simulink library "Vehicle_Inputs"  (R2025a)
settings: Solver=VariableStepAuto  StartTime=0.0  StopTime=10.0  RelTol=1e-3
values from neighbouring files (symbols this model uses):
  b = beta    [frameRotationXYextr.m]
libraries: Damper_Control_Axle2 x2, Vehicle_Outputs x2, simulink x2, Spring_Control_Axle2 x1, Damper_Control_Axle3 x1, Spring_Control_Axle3 x1, sim3dlib x1, Tire_Utilities x1
Description:
  | Simscape Vehicle Templates Library
  | 
  | Copyright 2018-2026 The MathWorks, Inc.
settings Model: Creator=smiller  LastModifiedBy=smiller
settings OptimizationCC: ReuseModelBlockBuffer=off
settings ModelReferenceCC: EnableRefExpFcnMdlSchedulingChecks=on
settings RTWCC: GPUComputeCapability=3.5

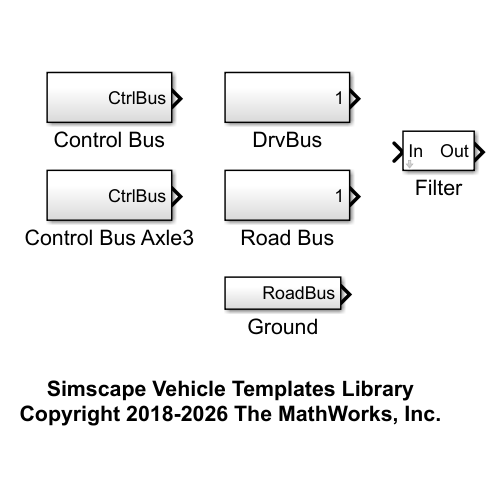
[thumbnail: Simulink's stored preview of the top-level diagram]
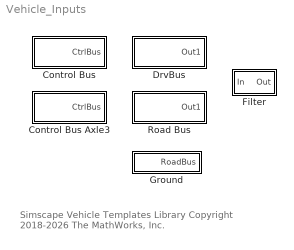
== system Vehicle_Inputs ==
  note: Simscape Vehicle Templates Library
      | Copyright 2018-2026 The MathWorks, Inc.
  Control Bus : Subsystem
  Control Bus Axle3 : Subsystem
  DrvBus : Subsystem
  Filter : Subsystem  mask(First-order lag supporting vector signals){b=b, x_initial=[0 0 0 0]}
      mask prompts: b "Filter time constant"; x_initial "Initial output"
      mask help: Models a lag of the form 1/(b*s+1) where s is the Laplace operator.
  Ground : Subsystem
  Road Bus : Subsystem

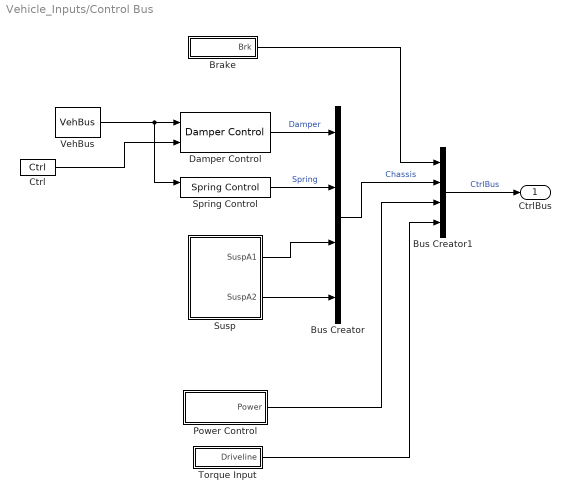
== system Vehicle_Inputs/Control Bus ==
  Brake : Subsystem  mask{brake_on_time=10}
      mask prompts: brake_on_time "Brake On Time (sec)"
      mask TypeOptions brake_on_time: Step/Time
  Bus Creator : BusCreator  Inputs=4
  Bus Creator1 : BusCreator  Inputs=4
  Ctrl : Damper_Control_Axle2/Ctrl  SystemSampleTime=-1  VariantActivationTime=update diagram  EmptyChoice=off  PassThrough=off  PassThroughVariantControl=(default)  EmptyChoiceVariantControl=(default)  AllowFlexibleInterface=on  Latency=0  AutoFrameSizeCalculation=off
  Damper Control : Damper_Control_Axle2/Damper Control  popup_damper_control_A1=Coefficient  popup_damper_control_A2=Coefficient
  Power Control : Subsystem
  Spring Control : Spring_Control_Axle2/Spring Control  VariantControl=Choice  popup_spring_control_A1=None  popup_gas_spring_A1=Stiff  popup_spring_control_A2=None  popup_gas_spring_A2=Stiff
      settings: AttributesFormatString=%<popup_spring_control>
  Susp : Subsystem
  Torque Input : Subsystem  mask{popup_torque_input=Low Torque, Rear}
      mask prompts: popup_torque_input "Maneuver Torque"
      mask init:
      | if (popup_torque_input == 1)
      |     torque_ra = 200*2*2*2;
      |     torque_fa = 0;
      | elseif (popup_torque_input == 2)
      |     torque_ra = 0;
      |     torque_fa = 200*2*2*2;
      | elseif (popup_torque_input == 3)
      |     torque_ra = 200*2;
      |     torque_fa = 0;
      | elseif (popup_torque_input == 4)
      |     torque_ra = 0;
      |     torque_fa = 200*2;
      | elseif (popup_torque_input == 5)
      |     torque_ra = 0;
      |     torque_fa = 0;
      | end
      mask TypeOptions popup_torque_input: Full Torque, Rear | Full Torque, Front | Low Torque, Rear | Low Torque, Front | None
  VehBus : Vehicle_Outputs/VehBus  SystemSampleTime=-1  VariantActivationTime=update diagram  EmptyChoice=off  PassThrough=off  PassThroughVariantControl=(default)  EmptyChoiceVariantControl=(default)  AllowFlexibleInterface=on  Latency=0  AutoFrameSizeCalculation=off
  CtrlBus : Outport  VectorParamsAs1DForOutWhenUnconnected=off
  wires:
  Power Control/1(Power) -> Bus Creator1/3
  Bus Creator/1 -> Bus Creator1/2  "Chassis"
  Torque Input/1(Driveline) -> Bus Creator1/4
  Brake/1(Brk) -> Bus Creator1/1
  Bus Creator1/1 -> CtrlBus/1  "CtrlBus"
  Susp/2(SuspA2) -> Bus Creator/4
  Susp/1(SuspA1) -> Bus Creator/3
  VehBus/1 -> Spring Control/1, Damper Control/1
  Damper Control/1 -> Bus Creator/1  "Damper"
  Spring Control/1 -> Bus Creator/2  "Spring"
  Ctrl/1 -> Damper Control/2

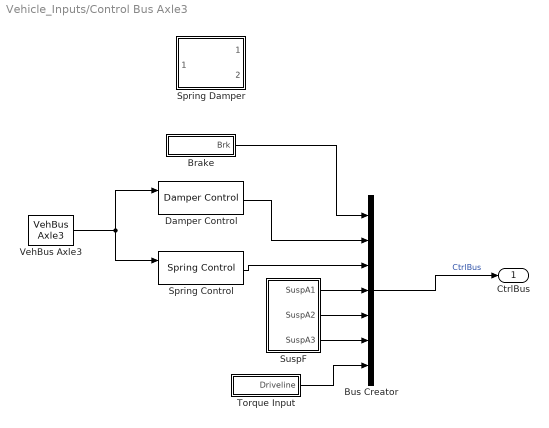
== system Vehicle_Inputs/Control Bus Axle3 ==
  Brake : Subsystem  mask{brake_on_time=10}
      mask prompts: brake_on_time "Brake On Time (sec)"
      mask TypeOptions brake_on_time: Step/Time
  Bus Creator : BusCreator  Inputs=7
  Damper Control : Damper_Control_Axle3/Damper Control  VariantControl=Choice  popup_damper_control_A1=None  popup_damper_control_A2=None  popup_damper_control_A3=None
      settings: AttributesFormatString=%<popup_damper_control>
  Spring Control : Spring_Control_Axle3/Spring Control  VariantControl=Choice  popup_spring_control_A1=None  popup_spring_control_A2=None  popup_spring_control_A3=None
      settings: AttributesFormatString=%<popup_spring_control>
  Spring Damper : Subsystem
  SuspF : Subsystem
  Torque Input : Subsystem  mask{popup_torque_input=Low Torque, Rear}
      mask prompts: popup_torque_input "Maneuver Torque"
      mask init: same as Vehicle_Inputs/Control Bus/Torque Input
      mask TypeOptions popup_torque_input: Full Torque, Rear | Full Torque, Front | Low Torque, Rear | Low Torque, Front | None
  VehBus Axle3 : Vehicle_Outputs/VehBus Axle3  SystemSampleTime=-1  VariantActivationTime=update diagram  EmptyChoice=off  PassThrough=off  PassThroughVariantControl=(default)  EmptyChoiceVariantControl=(default)  AllowFlexibleInterface=on  Latency=0  AutoFrameSizeCalculation=off
  CtrlBus : Outport  VectorParamsAs1DForOutWhenUnconnected=off
  wires:
  SuspF/3(SuspA3) -> Bus Creator/6
  SuspF/1(SuspA1) -> Bus Creator/4
  SuspF/2(SuspA2) -> Bus Creator/5
  Bus Creator/1 -> CtrlBus/1  "CtrlBus"
  Spring Control/1 -> Bus Creator/3
  Damper Control/1 -> Bus Creator/2
  Brake/1(Brk) -> Bus Creator/1
  Torque Input/1(Driveline) -> Bus Creator/7
  VehBus Axle3/1 -> Spring Control/1, Damper Control/1

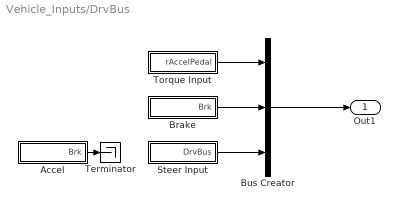
== system Vehicle_Inputs/DrvBus ==
  Accel : Subsystem  mask{brake_on_time=10}
      mask prompts: brake_on_time "Brake On Time (sec)"
      mask TypeOptions brake_on_time: Step/Time
  Brake : Subsystem  mask{brake_on_time=10}
      mask prompts: brake_on_time "Brake On Time (sec)"
      mask TypeOptions brake_on_time: Step/Time
  Bus Creator : BusCreator  Inputs=3
  Steer Input : Subsystem  mask{popup_steer_input=Sequence}
      mask prompts: popup_steer_input "Steer Input"
      mask TypeOptions popup_steer_input: Straight | Step | Sequence | Lane Change
  Terminator : Terminator
  Torque Input : Subsystem  mask{popup_torque_input=Full Torque}
      mask prompts: popup_torque_input "Maneuver Torque"
      mask init:
      | if (popup_torque_input == 1)
      |     rPedalValue = 1;
      | elseif (popup_torque_input == 2)
      |     rPedalValue = 0.25;
      | elseif (popup_torque_input == 3)
      |     rPedalValue = 0;
      | end
      mask TypeOptions popup_torque_input: Full Torque | Low Torque | None
  Out1 : Outport  VectorParamsAs1DForOutWhenUnconnected=off
  wires:
  Accel/1(Brk) -> Terminator/1
  Torque Input/1(rAccelPedal) -> Bus Creator/1
  Brake/1(Brk) -> Bus Creator/2
  Bus Creator/1 -> Out1/1
  Steer Input/1(DrvBus) -> Bus Creator/3

== system Vehicle_Inputs/Filter ==
  In : Inport
  Gain : Gain  Gain=1/b
  Integrator : Integrator  InitialCondition=x_initial*b
  Sum : Sum  Inputs=|+-  InputSameDT=on  SaturateOnIntegerOverflow=on  OutDataTypeStr=Inherit: Same as first input
  Out : Outport  VectorParamsAs1DForOutWhenUnconnected=off
  wires:
  Sum/1 -> Integrator/1
  In/1 -> Sum/1
  Integrator/1 -> Gain/1
  Gain/1 -> Sum/2, Out/1

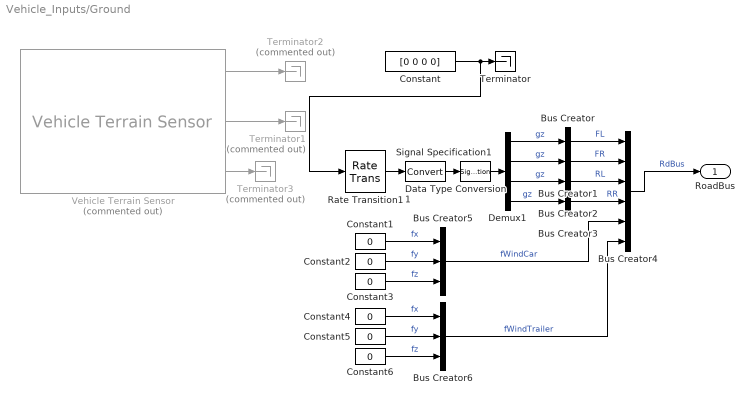
== system Vehicle_Inputs/Ground ==
  Bus Creator{,1..3} (4 alike) : BusCreator  Inputs=1
  Bus Creator4 : BusCreator  Inputs=6
  Bus Creator5 : BusCreator  Inputs=3
  Bus Creator6 : BusCreator  Inputs=3
  Constant : Constant  Value=[0 0 0 0]
  Constant{1..6} (6 alike) : Constant  Value=0
  Data Type Conversion1 : DataTypeConversion  SaturateOnIntegerOverflow=off  RndMeth=Floor
  Demux1 : Demux
  Rate Transition1 : RateTransition
  Signal Specification1 : SignalSpecification  Unit=m
  Terminator : Terminator
  Terminator1 : Terminator  Commented=on
  Terminator2 : Terminator  Commented=on
  Terminator3 : Terminator  Commented=on
  Vehicle Terrain Sensor : sim3dlib/Vehicle Terrain Sensor  Commented=on  ActorTag=SimulinkActor1  VehExtEn=Constant  TireRadiiExt=Constant  VehCntrLngthVal=0  TireRadiiVal=.55  VehRayLngth=5  LfRayLngth=5  RfRayLngth=5  LrRayLngth=5  RrRayLngth=5  VehRayOffset=0  LfRayOffset=0  RfRayOffset=0  LrRayOffset=0  RrRayOffset=0  VehEn=on  LfEn=on  RfEn=on  LrEn=on  RrEn=on  DbgEn=off  Ts=0.06  aMode=aMode
  RoadBus : Outport  VectorParamsAs1DForOutWhenUnconnected=off
  wires:
  Constant4/1 -> Bus Creator6/1  "fx"
  Constant5/1 -> Bus Creator6/2  "fy"
  Constant6/1 -> Bus Creator6/3  "fz"
  Bus Creator6/1 -> Bus Creator4/6  "fWindTrailer"
  Bus Creator5/1 -> Bus Creator4/5  "fWindCar"
  Constant3/1 -> Bus Creator5/3  "fz"
  Constant2/1 -> Bus Creator5/2  "fy"
  Constant1/1 -> Bus Creator5/1  "fx"
  Vehicle Terrain Sensor/3 -> Terminator3/1
  Signal Specification1/1 -> Demux1/1
  Bus Creator2/1 -> Bus Creator4/3  "RL"
  Bus Creator3/1 -> Bus Creator4/4  "RR"
  Demux1/4 -> Bus Creator3/1  "gz"
  Demux1/1 -> Bus Creator/1  "gz"
  Demux1/2 -> Bus Creator1/1  "gz"
  Demux1/3 -> Bus Creator2/1  "gz"
  Bus Creator/1 -> Bus Creator4/1  "FL"
  Bus Creator1/1 -> Bus Creator4/2  "FR"
  Bus Creator4/1 -> RoadBus/1  "RdBus"
  Rate Transition1/1 -> Data Type Conversion1/1
  Data Type Conversion1/1 -> Signal Specification1/1
  Vehicle Terrain Sensor/1 -> Terminator2/1
  Vehicle Terrain Sensor/2 -> Terminator1/1
  Constant/1 -> Terminator/1, Rate Transition1/1

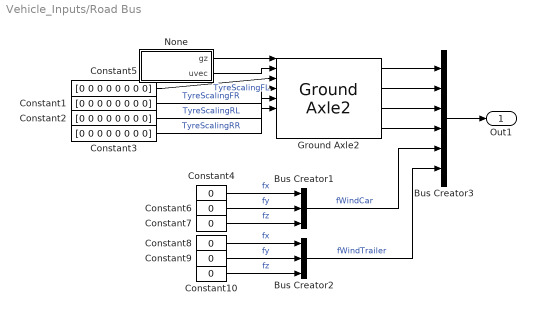
== system Vehicle_Inputs/Road Bus ==
  Bus Creator1 : BusCreator  Inputs=3
  Bus Creator2 : BusCreator  Inputs=3
  Bus Creator3 : BusCreator  Inputs=6
  Constant{1..3,5} (4 alike) : Constant  Value=[0 0 0 0 0 0 0 0]
  Constant{4,6..10} (6 alike) : Constant  Value=0
  Ground Axle2 : Tire_Utilities/Ground Axle2  SystemSampleTime=-1  VariantActivationTime=update diagram  EmptyChoice=off  PassThrough=off  PassThroughVariantControl=(default)  EmptyChoiceVariantControl=(default)  AllowFlexibleInterface=on  Latency=0  AutoFrameSizeCalculation=off
  None : Subsystem  VariantControl=None
  Out1 : Outport  VectorParamsAs1DForOutWhenUnconnected=off
  wires:
  Bus Creator3/1 -> Out1/1
  Ground Axle2/4 -> Bus Creator3/4
  Ground Axle2/3 -> Bus Creator3/3
  Ground Axle2/2 -> Bus Creator3/2
  Ground Axle2/1 -> Bus Creator3/1
  Bus Creator2/1 -> Bus Creator3/6  "fWindTrailer"
  Constant9/1 -> Bus Creator2/2  "fy"
  Constant10/1 -> Bus Creator2/3  "fz"
  Constant8/1 -> Bus Creator2/1  "fx"
  Bus Creator1/1 -> Bus Creator3/5  "fWindCar"
  Constant4/1 -> Bus Creator1/1  "fx"
  Constant7/1 -> Bus Creator1/3  "fz"
  Constant6/1 -> Bus Creator1/2  "fy"
  Constant3/1 -> Ground Axle2/6  "TyreScalingRR"
  Constant2/1 -> Ground Axle2/5  "TyreScalingRL"
  Constant1/1 -> Ground Axle2/4  "TyreScalingFR"
  Constant5/1 -> Ground Axle2/3  "TyreScalingFL"
  None/2(uvec) -> Ground Axle2/2
  None/1(gz) -> Ground Axle2/1

== system Vehicle_Inputs/Control Bus/Brake ==
  Bus Creator : BusCreator  Inputs=4
  Demux : Demux
  Step : Step  Time=brake_on_time  After=[1 1 1 1]  SampleTime=0  ZeroCross=off
  Brk : Outport  VectorParamsAs1DForOutWhenUnconnected=off
  wires:
  Step/1 -> Demux/1
  Bus Creator/1 -> Brk/1  "Brakes"
  Demux/3 -> Bus Creator/3  "pBrakeRL"
  Demux/4 -> Bus Creator/4  "pBrakeRR"
  Demux/1 -> Bus Creator/1  "pBrakeFL"
  Demux/2 -> Bus Creator/2  "pBrakeFR"

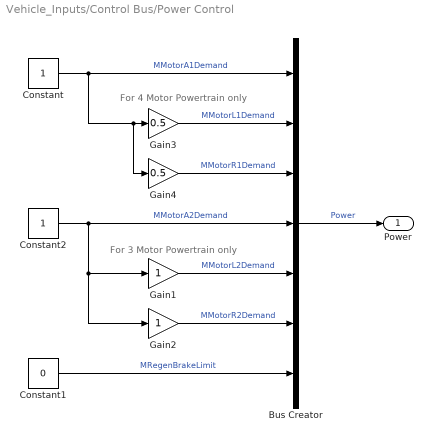
== system Vehicle_Inputs/Control Bus/Power Control ==
  note: For 4 Motor Powertrain only
  note: For 3 Motor Powertrain only
  Bus Creator : BusCreator  Inputs=7
  Constant : Constant
  Constant1 : Constant  Value=0
  Constant2 : Constant
  Gain1 : Gain
  Gain2 : Gain
  Gain3 : Gain  Gain=0.5
  Gain4 : Gain  Gain=0.5
  Power : Outport  VectorParamsAs1DForOutWhenUnconnected=off
  wires:
  Bus Creator/1 -> Power/1  "Power"
  Constant2/1 -> Gain2/1, Gain1/1, Bus Creator/4  "MMotorA2Demand"
  Constant/1 -> Gain4/1, Gain3/1, Bus Creator/1  "MMotorA1Demand"
  Constant1/1 -> Bus Creator/7  "MRegenBrakeLimit"
  Gain1/1 -> Bus Creator/5  "MMotorL2Demand"
  Gain2/1 -> Bus Creator/6  "MMotorR2Demand"
  Gain3/1 -> Bus Creator/2  "MMotorL1Demand"
  Gain4/1 -> Bus Creator/3  "MMotorR1Demand"

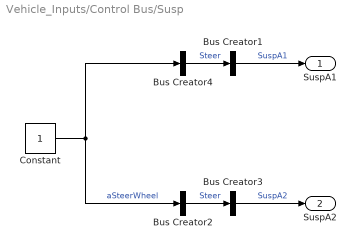
== system Vehicle_Inputs/Control Bus/Susp ==
  Bus Creator{1..4} (4 alike) : BusCreator  Inputs=1
  Constant : Constant
  SuspA1 : Outport  VectorParamsAs1DForOutWhenUnconnected=off
  SuspA2 : Outport  Port=2  VectorParamsAs1DForOutWhenUnconnected=off
  wires:
  Constant/1 -> Bus Creator2/1, Bus Creator4/1  "aSteerWheel"
  Bus Creator1/1 -> SuspA1/1  "SuspA1"
  Bus Creator3/1 -> SuspA2/1  "SuspA2"
  Bus Creator2/1 -> Bus Creator3/1  "Steer"
  Bus Creator4/1 -> Bus Creator1/1  "Steer"

== system Vehicle_Inputs/Control Bus/Torque Input ==
  Bus Creator : BusCreator  Inputs=2
  Front Torque Enable : Gain
  Rear Torque Enable : Gain
  Torque Front : Subsystem  mask{on_time=1, off_time=10, torque_value=torque_fa}
      mask prompts: on_time "On Time (s)"; off_time "Off Time (s)"; torque_value "Torque Value (N*m)"
      mask TypeOptions on_time: Step On/Time
      mask TypeOptions off_time: Step Off/Time
      mask TypeOptions torque_value: Step Height/Gain
  Torque Rear : Subsystem  mask{on_time=1, off_time=10, torque_value=torque_ra}
      mask prompts: on_time "On Time (s)"; off_time "Off Time (s)"; torque_value "Torque Value (N*m)"
      mask TypeOptions on_time: Step On/Time
      mask TypeOptions off_time: Step Off/Time
      mask TypeOptions torque_value: Step Height/Gain
  Driveline : Outport  VectorParamsAs1DForOutWhenUnconnected=off
  wires:
  Torque Rear/1(MMotorRDemand) -> Rear Torque Enable/1
  Bus Creator/1 -> Driveline/1  "Driveline"
  Front Torque Enable/1 -> Bus Creator/1  "MMotorA1Demand"
  Rear Torque Enable/1 -> Bus Creator/2  "MMotorA2Demand"
  Torque Front/1(MMotorRDemand) -> Front Torque Enable/1

== system Vehicle_Inputs/Control Bus Axle3/Brake ==
  Bus Creator : BusCreator  Inputs=6
  Demux : Demux  Outputs=6
  Step : Step  Time=brake_on_time  After=[1 1 1 1 1 1]  SampleTime=0  ZeroCross=off
  Brk : Outport  VectorParamsAs1DForOutWhenUnconnected=off
  wires:
  Demux/6 -> Bus Creator/6  "pBrakeR3"
  Demux/5 -> Bus Creator/5  "pBrakeL3"
  Demux/2 -> Bus Creator/2  "pBrakeR1"
  Demux/1 -> Bus Creator/1  "pBrakeL1"
  Demux/4 -> Bus Creator/4  "pBrakeR2"
  Demux/3 -> Bus Creator/3  "pBrakeL2"
  Bus Creator/1 -> Brk/1  "Brakes"
  Step/1 -> Demux/1

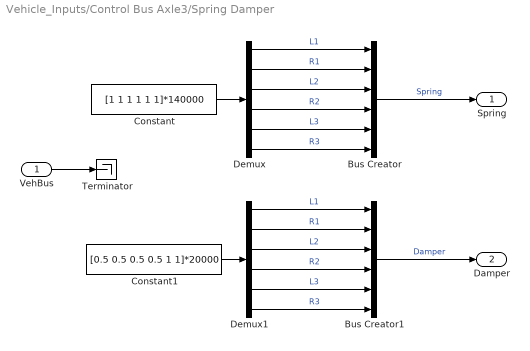
== system Vehicle_Inputs/Control Bus Axle3/Spring Damper ==
  VehBus : Inport
  Bus Creator : BusCreator  Inputs=6
  Bus Creator1 : BusCreator  Inputs=6
  Constant : Constant  Value=[1 1 1 1 1 1]*140000
  Constant1 : Constant  Value=[0.5 0.5 0.5 0.5 1 1]*20000
  Demux : Demux  Outputs=6
  Demux1 : Demux  Outputs=6
  Terminator : Terminator
  Spring : Outport  VectorParamsAs1DForOutWhenUnconnected=off
  Damper : Outport  Port=2  VectorParamsAs1DForOutWhenUnconnected=off
  wires:
  Demux1/6 -> Bus Creator1/6  "R3"
  Demux1/5 -> Bus Creator1/5  "L3"
  Demux/6 -> Bus Creator/6  "R3"
  Demux/5 -> Bus Creator/5  "L3"
  Constant/1 -> Demux/1
  Demux/3 -> Bus Creator/3  "L2"
  Demux/4 -> Bus Creator/4  "R2"
  Demux/1 -> Bus Creator/1  "L1"
  Demux/2 -> Bus Creator/2  "R1"
  Demux1/2 -> Bus Creator1/2  "R1"
  Demux1/1 -> Bus Creator1/1  "L1"
  Demux1/4 -> Bus Creator1/4  "R2"
  Demux1/3 -> Bus Creator1/3  "L2"
  Constant1/1 -> Demux1/1
  Bus Creator1/1 -> Damper/1  "Damper"
  Bus Creator/1 -> Spring/1  "Spring"
  VehBus/1 -> Terminator/1

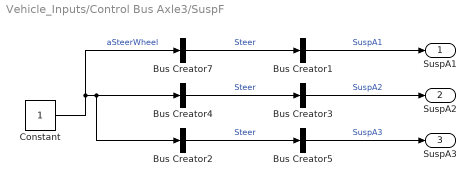
== system Vehicle_Inputs/Control Bus Axle3/SuspF ==
  Bus Creator{1..5,7} (6 alike) : BusCreator  Inputs=1
  Constant : Constant
  SuspA1 : Outport  VectorParamsAs1DForOutWhenUnconnected=off
  SuspA2 : Outport  Port=2  VectorParamsAs1DForOutWhenUnconnected=off
  SuspA3 : Outport  Port=3  VectorParamsAs1DForOutWhenUnconnected=off
  wires:
  Constant/1 -> Bus Creator4/1, Bus Creator2/1, Bus Creator7/1  "aSteerWheel"
  Bus Creator2/1 -> Bus Creator5/1  "Steer"
  Bus Creator4/1 -> Bus Creator3/1  "Steer"
  Bus Creator7/1 -> Bus Creator1/1  "Steer"
  Bus Creator5/1 -> SuspA3/1  "SuspA3"
  Bus Creator1/1 -> SuspA1/1  "SuspA1"
  Bus Creator3/1 -> SuspA2/1  "SuspA2"

== system Vehicle_Inputs/Control Bus Axle3/Torque Input ==
  Bus Creator : BusCreator  Inputs=2
  Front Torque Enable : Gain
  Rear Torque Enable : Gain
  Torque Front : Subsystem  mask{on_time=1, off_time=10, torque_value=torque_fa}
      mask prompts: on_time "On Time (s)"; off_time "Off Time (s)"; torque_value "Torque Value (N*m)"
      mask TypeOptions on_time: Step On/Time
      mask TypeOptions off_time: Step Off/Time
      mask TypeOptions torque_value: Step Height/Gain
  Torque Rear : Subsystem  mask{on_time=1, off_time=10, torque_value=torque_ra}
      mask prompts: on_time "On Time (s)"; off_time "Off Time (s)"; torque_value "Torque Value (N*m)"
      mask TypeOptions on_time: Step On/Time
      mask TypeOptions off_time: Step Off/Time
      mask TypeOptions torque_value: Step Height/Gain
  Driveline : Outport  VectorParamsAs1DForOutWhenUnconnected=off
  wires:
  Torque Front/1(MMotorRDemand) -> Front Torque Enable/1
  Rear Torque Enable/1 -> Bus Creator/2  "MMotorA2Demand"
  Front Torque Enable/1 -> Bus Creator/1  "MMotorA1Demand"
  Bus Creator/1 -> Driveline/1  "Driveline"
  Torque Rear/1(MMotorRDemand) -> Rear Torque Enable/1

== system Vehicle_Inputs/DrvBus/Accel ==
  Step : Step  Time=brake_on_time  After=[1 1 1 1]  SampleTime=0  ZeroCross=off
  Brk : Outport  VectorParamsAs1DForOutWhenUnconnected=off
  wires:
  Step/1 -> Brk/1  "rBrakePedal"

== system Vehicle_Inputs/DrvBus/Brake ==
  Step : Step  Time=brake_on_time  SampleTime=0  ZeroCross=off
  Brk : Outport  VectorParamsAs1DForOutWhenUnconnected=off
  wires:
  Step/1 -> Brk/1  "rBrakePedal"

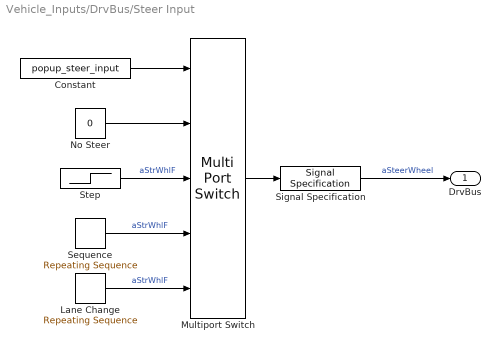
== system Vehicle_Inputs/DrvBus/Steer Input ==
  Constant : Constant  Value=popup_steer_input
  Lane Change : simulink/Sources/Repeating Sequence  rep_seq_t=[0 10 10.5 11.5 12 13 13.5 20]  rep_seq_y=[0 0 1 1 -1 -1 0 0]*5*pi/180
  Multiport Switch : MultiPortSwitch  Inputs=4  SaturateOnIntegerOverflow=off  InputSameDT=off
  No Steer : Constant  Value=0
  Sequence : simulink/Sources/Repeating Sequence  rep_seq_t=[0 1 2 3 4 5]  rep_seq_y=[0 0 -1 1 0 0]*5*pi/180
  Signal Specification : SignalSpecification  Unit=rad
  Step : Step  Time=5  After=5*pi/180  SampleTime=0  ZeroCross=off
      settings: AttributesFormatString=%<After> @ %<Time> sec
  DrvBus : Outport  VectorParamsAs1DForOutWhenUnconnected=off
  wires:
  Multiport Switch/1 -> Signal Specification/1
  Lane Change/1 -> Multiport Switch/5  "aStrWhlF"
  Signal Specification/1 -> DrvBus/1  "aSteerWheel"
  No Steer/1 -> Multiport Switch/2
  Step/1 -> Multiport Switch/3  "aStrWhlF"
  Constant/1 -> Multiport Switch/1
  Sequence/1 -> Multiport Switch/4  "aStrWhlF"

== system Vehicle_Inputs/DrvBus/Torque Input ==
  Torque Front : Subsystem  mask{on_time=1, off_time=10, rPedalValue=rPedalValue}
      mask prompts: on_time "On Time (s)"; off_time "Off Time (s)"; rPedalValue "Torque Value (N*m)"
      mask TypeOptions on_time: Step On/Time
      mask TypeOptions off_time: Step Off/Time
      mask TypeOptions rPedalValue: Gain/Gain
  rAccelPedal : Outport  VectorParamsAs1DForOutWhenUnconnected=off
  wires:
  Torque Front/1(rAccelPedal) -> rAccelPedal/1  "rAccelPedal"

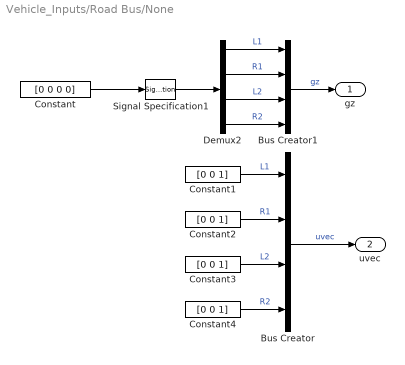
== system Vehicle_Inputs/Road Bus/None ==
  Bus Creator : BusCreator  Inputs=4
  Bus Creator1 : BusCreator  Inputs=4
  Constant : Constant  Value=[0 0 0 0]
  Constant{1..4} (4 alike) : Constant  Value=[0 0 1]
  Demux2 : Demux
  Signal Specification1 : SignalSpecification  Unit=m
  gz : Outport  VectorParamsAs1DForOutWhenUnconnected=off
  uvec : Outport  Port=2  VectorParamsAs1DForOutWhenUnconnected=off
  wires:
  Constant/1 -> Signal Specification1/1
  Demux2/1 -> Bus Creator1/1  "L1"
  Signal Specification1/1 -> Demux2/1
  Bus Creator1/1 -> gz/1  "gz"
  Demux2/2 -> Bus Creator1/2  "R1"
  Demux2/4 -> Bus Creator1/4  "R2"
  Demux2/3 -> Bus Creator1/3  "L2"
  Constant3/1 -> Bus Creator/3  "L2"
  Constant2/1 -> Bus Creator/2  "R1"
  Constant1/1 -> Bus Creator/1  "L1"
  Constant4/1 -> Bus Creator/4  "R2"
  Bus Creator/1 -> uvec/1  "uvec"

== system Vehicle_Inputs/Control Bus/Torque Input/Torque Front ==
  Gain : Gain
  Rate Limiter : RateLimiter  RisingSlewLimit=300  FallingSlewLimit=-300  SampleTimeMode=inherited
  Step Height : Gain  Gain=torque_value
  Step Off : Step  Time=off_time  After=-1  SampleTime=0  ZeroCross=off
  Step On : Step  Time=on_time  SampleTime=0  ZeroCross=off
  Sum : Sum  Inputs=|++
  MMotorRDemand : Outport  VectorParamsAs1DForOutWhenUnconnected=off
  wires:
  Step Height/1 -> Rate Limiter/1
  Rate Limiter/1 -> Gain/1
  Step On/1 -> Sum/1
  Sum/1 -> Step Height/1
  Step Off/1 -> Sum/2
  Gain/1 -> MMotorRDemand/1  "MMotorRDemand"

== system Vehicle_Inputs/Control Bus/Torque Input/Torque Rear ==
  Gain : Gain
  Rate Limiter : RateLimiter  RisingSlewLimit=300  FallingSlewLimit=-300  SampleTimeMode=inherited
  Step Height : Gain  Gain=torque_value
  Step Off : Step  Time=off_time  After=-1  SampleTime=0  ZeroCross=off
  Step On : Step  Time=on_time  SampleTime=0  ZeroCross=off
  Sum : Sum  Inputs=|++
  MMotorRDemand : Outport  VectorParamsAs1DForOutWhenUnconnected=off
  wires:
  Gain/1 -> MMotorRDemand/1  "MMotorRDemand"
  Step Off/1 -> Sum/2
  Sum/1 -> Step Height/1
  Step On/1 -> Sum/1
  Rate Limiter/1 -> Gain/1
  Step Height/1 -> Rate Limiter/1

== system Vehicle_Inputs/Control Bus Axle3/Torque Input/Torque Front ==
  Gain : Gain
  Rate Limiter : RateLimiter  RisingSlewLimit=300  FallingSlewLimit=-300  SampleTimeMode=inherited
  Step Height : Gain  Gain=torque_value
  Step Off : Step  Time=off_time  After=-1  SampleTime=0  ZeroCross=off
  Step On : Step  Time=on_time  SampleTime=0  ZeroCross=off
  Sum : Sum  Inputs=|++
  MMotorRDemand : Outport  VectorParamsAs1DForOutWhenUnconnected=off
  wires:
  Gain/1 -> MMotorRDemand/1  "MMotorRDemand"
  Step Off/1 -> Sum/2
  Sum/1 -> Step Height/1
  Step On/1 -> Sum/1
  Rate Limiter/1 -> Gain/1
  Step Height/1 -> Rate Limiter/1

== system Vehicle_Inputs/Control Bus Axle3/Torque Input/Torque Rear ==
  Gain : Gain
  Rate Limiter : RateLimiter  RisingSlewLimit=300  FallingSlewLimit=-300  SampleTimeMode=inherited
  Step Height : Gain  Gain=torque_value
  Step Off : Step  Time=off_time  After=-1  SampleTime=0  ZeroCross=off
  Step On : Step  Time=on_time  SampleTime=0  ZeroCross=off
  Sum : Sum  Inputs=|++
  MMotorRDemand : Outport  VectorParamsAs1DForOutWhenUnconnected=off
  wires:
  Step Height/1 -> Rate Limiter/1
  Rate Limiter/1 -> Gain/1
  Step On/1 -> Sum/1
  Sum/1 -> Step Height/1
  Step Off/1 -> Sum/2
  Gain/1 -> MMotorRDemand/1  "MMotorRDemand"

== system Vehicle_Inputs/DrvBus/Torque Input/Torque Front ==
  Gain : Gain  Gain=rPedalValue
  Step Off : Step  Time=off_time  After=-1  SampleTime=0  ZeroCross=off
  Step On : Step  Time=on_time  SampleTime=0  ZeroCross=off
  Sum : Sum  Inputs=|++
  rAccelPedal : Outport  VectorParamsAs1DForOutWhenUnconnected=off
  wires:
  Gain/1 -> rAccelPedal/1  "rAccelPedal"
  Step On/1 -> Sum/1
  Step Off/1 -> Sum/2
  Sum/1 -> Gain/1
